simulink model "sf_spectrum_analyzer"  (R2025b)
settings: Solver=ode5  StartTime=0.0  StopTime=Inf  FixedStep=1e-4  MaxStep=1e-4  RelTol=1e-3  EnableMultiTasking=on
settings Model: Creator=The MathWorks, Inc.  LastModifiedBy=The MathWorks, Inc.
settings SolverCC: AlgebraicLoopSolver=TrustRegion
settings DataIOCC: SaveFormat=Array  ReturnWorkspaceOutputs=off
settings OptimizationCC: ReuseModelBlockBuffer=off  ExpressionDepthLimit=2147483647.0  InitFltsAndDblsToZero=on  EfficientMapNaN2IntZero=off  LifeSpan=1  EfficientTunableParamExpr=on
settings DebuggingCC: UnderspecifiedInitializationDetection=Classic  MergeDetectMultiDrivingBlocksExec=none  SolverPrmCheckMsg=warning  FcnCallInpInsideContextMsg=warning  UnconnectedInputMsg=warning  UnconnectedOutputMsg=warning  UnconnectedLineMsg=warning  StateNameClashWarn=warning  SFUnexpectedBacktrackingDiag=warning  SFNoUnconditionalDefaultTransitionDiag=warning  SFExecutionAtInitializationDiag=none  ArithmeticOperatorsInVariantConditions=warning
settings HardwareCC: ProdBitPerPointer=32.0  ProdBitPerSizeT=32.0  ProdBitPerPtrDiffT=32.0  ProdLargestAtomicFloat=None  ProdIntDivRoundTo=Undefined  ProdEndianess=Unspecified  ProdWordSize=32.0  ProdHWDeviceType=32-bit Generic
settings ModelReferenceCC: EnableRefExpFcnMdlSchedulingChecks=on  PropagateSignalLabelsOutOfModel=off
settings SFSimCC: SimUseLocalCustomCode=off  SimParseCustomCode=off  MATLABDynamicMemAlloc=off  CustomCodeUndefinedFunction=UseInterfaceOnly
settings RTWCC: SystemTargetFile=ert.tlc  TemplateMakefile=ert_default_tmf  GenerateReport=on  RTWUseLocalCustomCode=off  IncludeHyperlinkInReport=on  LaunchReport=on  GenerateTraceInfo=on  GenerateTraceReport=on  GenerateTraceReportSl=on  GenerateTraceReportSf=on  GenerateTraceReportEml=on  GPUComputeCapability=3.5  DLArmComputeVersion=19.05  Description=Real-Time Workshop Embedded Coder (no auto configuration)
settings CodeAppCC: IgnoreCustomStorageClasses=off  CustomSymbolStrType=$N$R$M  StateflowObjectComments=on  InternalIdentifier=Classic
settings ERTTargetCC: InlinedParameterPlacement=Hierarchical  ERTCustomFileTemplate=example_file_process.tlc  ConvertIfToSwitch=off  SuppressUnreachableDefaultCases=off  MultiwordLength=2048.0  GenerateSampleERTMain=on  SupportContinuousTime=on
settings ConfigComp: CovMetricSettings=dw  CovSaveCumulativeToWorkspaceVar=on  CovSaveSingleToWorkspaceVar=on  CovExternalEMLEnable=off  CovSFcnEnable=off

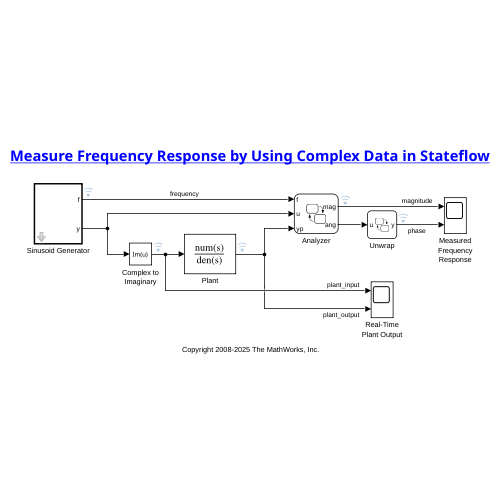
[thumbnail: Simulink's stored preview of the top-level diagram]
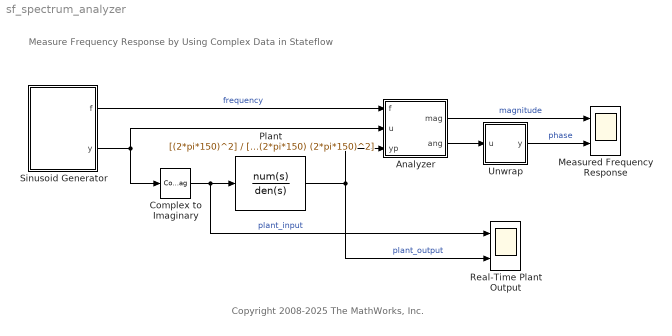
== system sf_spectrum_analyzer ==
  note: Copyright 2008-2025 The MathWorks, Inc.
  note: Measure Frequency Response by Using Complex Data in Stateflow
  Analyzer : Stateflow chart  TreatAsAtomicUnit=on
  Complex to Imaginary : ComplexToRealImag  Output=Imag
  Measured Frequency Response : Scope  NumInputPorts=2
      settings: TimeSpan=21  ActiveDisplayYMinimum=-0.21723  ActiveDisplayYMaximum=1.95511
  Plant : TransferFcn  Numerator=[(2*pi*150)^2]  Denominator=[1 2*0.3*(2*pi*150) (2*pi*150)^2]
  Real-Time Plant Output : Scope  NumInputPorts=2
      settings: TimeSpan=21  ActiveDisplayYMinimum=-1.2  ActiveDisplayYMaximum=1.2
  Sinusoid Generator : Subsystem  TreatAsAtomicUnit=on  mask{fstart=10, fstop=1000, fstep=10, delay=0.2}
      mask prompts: fstart "Initial frequency"; fstop "Stop frequency"; fstep "Step frequency"; delay "Delay at each frequency"
      mask help: Outputs a signal with constantly increasing frequency
  Unwrap : Stateflow chart  TreatAsAtomicUnit=on
  wires:
  Complex to Imaginary/1 -> Plant/1, Real-Time Plant Output/1  "plant_input"
  Plant/1 -> Analyzer/3(yp), Real-Time Plant Output/2  "plant_output"
  Analyzer/1(mag) -> Measured Frequency Response/1  "magnitude"
  Analyzer/2(ang) -> Unwrap/1(u)
  Sinusoid Generator/2(y) -> Complex to Imaginary/1, Analyzer/2(u)
  Sinusoid Generator/1(f) -> Analyzer/1(f)  "frequency"
  Unwrap/1(y) -> Measured Frequency Response/2  "phase"

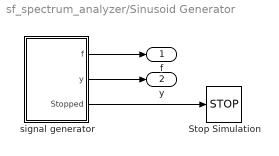
== system sf_spectrum_analyzer/Sinusoid Generator ==
  Stop Simulation : Stop
  signal generator : Stateflow chart  TreatAsAtomicUnit=on
  f : Outport  VectorParamsAs1DForOutWhenUnconnected=off
  y : Outport  Port=2  VectorParamsAs1DForOutWhenUnconnected=off
  wires:
  signal generator/2(y) -> y/1
  signal generator/1(f) -> f/1
  signal generator/3(" Stopped") -> Stop Simulation/1

== stateflow chart sf_spectrum_analyzer/Sinusoid Generator/signal generator ==
  state Generate
    en, du:
    t = temporalCount(sec);
    yprev = y;
    y = exp(2*pi*f*t*1i);
  state Stopped
  (default) -> Generate : {
      | f = fstart;
      | y = 0j;
      | }
  (junction 24) -> Generate
  Generate -> (junction 10) : [after(delay,sec) && imag(yprev) <= 0 && imag(y) > 0]
      | {
      | f = f + fstep;
      | }
  (junction 10) -> (junction 24) [order 2]
  (junction 10) -> Stopped [order 1] : [f > fstop]
  data: delay parameter double; f output; y output; yprev local; fstep parameter double; fstart parameter double; fstop parameter double; Stopped output boolean; t local

== stateflow chart sf_spectrum_analyzer/Analyzer ==
  state Analyze
    en:
    y = 0i; yn = 0i;
    du:
    y = y + u.*yp;
    yn = yn + u.*imag(u);
  (default) -> Analyze
  Analyze -> Analyze : [hasChanged(f)]
      | {
      | mag = abs(y)/abs(yn);
      | ang = -angle(y) + pi/2;
      | }
  data: f input; mag output; ang output; u input; y local; yn local; yp input

== stateflow chart sf_spectrum_analyzer/Unwrap ==
  state Update
    en, du:
    y = u+offset;
    uprev = u;
  (default) -> Update : {offset = 0;}
  Update -> Update [order 1] : [u-uprev > pi]
      | {offset = offset - 2*pi;}
  Update -> Update [order 2] : [u-uprev < -pi]
      | {offset = offset + 2*pi;}
  data: u input; y output; offset local; uprev local
